simulink model "elp_elec_env"  (R2026b)
settings: Solver=VariableStepAuto
undefined symbols (not defined in the file or in its folder): P, Ts
libraries: simulink x1
settings Model: Creator=aomar  LastModifiedBy=aomar

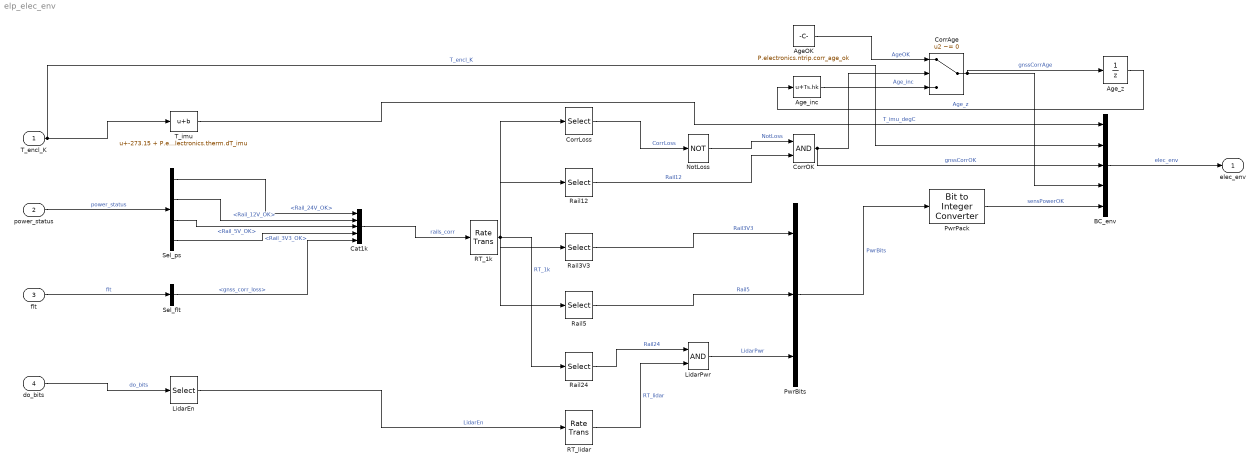
== system elp_elec_env ==
  T_encl_K : Inport  OutDataTypeStr=double  SampleTime=Ts.hk
  power_status : Inport  Port=2  OutDataTypeStr=Bus: Bus_PowerStatus  SampleTime=Ts.base
  flt : Inport  Port=3  OutDataTypeStr=Bus: Bus_FaultInject  SampleTime=Ts.base
  do_bits : Inport  Port=4  OutDataTypeStr=boolean  PortDimensions=32  SampleTime=Ts.ctrl
  AgeOK : Constant  Value=P.electronics.ntrip.corr_age_ok  OutDataTypeStr=double  SampleTime=Ts.hk
  Age_inc : Bias  Bias=Ts.hk  SaturateOnIntegerOverflow=off
  Age_z : UnitDelay  InitialCondition=P.electronics.ntrip.corr_age_ok  SampleTime=Ts.hk
  BC_env : BusCreator  Inputs=5  OutDataTypeStr=Bus: Bus_ElecEnv  NonVirtualBus=on
      settings: InheritFromInputs=off
  Cat1k : Concatenate  NumInputs=5
  CorrAge : Switch  Criteria=u2 ~= 0  SaturateOnIntegerOverflow=off  InputSameDT=off
  CorrLoss : Selector  InputPortWidth=5  IndexOptions=Index vector (dialog)  Indices=5  OutputSizes=1
  CorrOK : Logic  AllPortsSameDT=off  OutDataTypeStr=boolean
  LidarEn : Selector  InputPortWidth=32  IndexOptions=Index vector (dialog)  Indices=1 + P.electronics.do.lidar_pwr_en  OutputSizes=1
  LidarPwr : Logic  AllPortsSameDT=off  OutDataTypeStr=boolean
  NotLoss : Logic  Operator=NOT  Inputs=1  AllPortsSameDT=off  OutDataTypeStr=boolean
  PwrBits : Concatenate  NumInputs=3
  PwrPack : simulink/Logic and Bit Operations/Bit to Integer Converter  nbits=3  bitOrder=LSB first  signedOutputValues=Unsigned  outDtype=uint8  outDtypeSigned=Inherit via internal rule
      settings: LibrarySourceBlock=|
      | commutil2/Bit to Integer
      | Converter
  RT_1k : RateTransition  InitialCondition=false  OutPortSampleTime=Ts.hk
  RT_lidar : RateTransition  InitialCondition=false  OutPortSampleTime=Ts.hk
  Rail12 : Selector  InputPortWidth=5  IndexOptions=Index vector (dialog)  Indices=2  OutputSizes=1
  Rail24 : Selector  InputPortWidth=5  IndexOptions=Index vector (dialog)  Indices=1  OutputSizes=1
  Rail3V3 : Selector  InputPortWidth=5  IndexOptions=Index vector (dialog)  Indices=4  OutputSizes=1
  Rail5 : Selector  InputPortWidth=5  IndexOptions=Index vector (dialog)  Indices=3  OutputSizes=1
  Sel_flt : BusSelector  OutputSignals=gnss_corr_loss
  Sel_ps : BusSelector  OutputSignals=Rail_24V_OK,Rail_12V_OK,Rail_5V_OK,Rail_3V3_OK
  T_imu : Bias  Bias=-273.15 + P.electronics.therm.dT_imu  SaturateOnIntegerOverflow=off
  elec_env : Outport  OutDataTypeStr=Bus: Bus_ElecEnv
  wires:
  T_encl_K/1 -> T_imu/1, BC_env/2  "T_encl_K"
  power_status/1 -> Sel_ps/1  "power_status"
  flt/1 -> Sel_flt/1  "flt"
  do_bits/1 -> LidarEn/1  "do_bits"
  Sel_ps/1 -> Cat1k/1  "<Rail_24V_OK>"
  Sel_ps/2 -> Cat1k/2  "<Rail_12V_OK>"
  Sel_ps/3 -> Cat1k/3  "<Rail_5V_OK>"
  Sel_ps/4 -> Cat1k/4  "<Rail_3V3_OK>"
  Sel_flt/1 -> Cat1k/5  "<gnss_corr_loss>"
  T_imu/1 -> BC_env/1  "T_imu_degC"
  LidarEn/1 -> RT_lidar/1  "LidarEn"
  Cat1k/1 -> RT_1k/1  "rails_corr"
  RT_1k/1 -> Rail24/1, CorrLoss/1, Rail5/1, Rail12/1, Rail3V3/1  "RT_1k"
  CorrLoss/1 -> NotLoss/1  "CorrLoss"
  Rail12/1 -> CorrOK/2  "Rail12"
  Rail3V3/1 -> PwrBits/1  "Rail3V3"
  Rail5/1 -> PwrBits/2  "Rail5"
  Rail24/1 -> LidarPwr/1  "Rail24"
  RT_lidar/1 -> LidarPwr/2  "RT_lidar"
  NotLoss/1 -> CorrOK/1  "NotLoss"
  LidarPwr/1 -> PwrBits/3  "LidarPwr"
  PwrBits/1 -> PwrPack/1  "PwrBits"
  AgeOK/1 -> CorrAge/1  "AgeOK"
  CorrOK/1 -> CorrAge/2, BC_env/3  "gnssCorrOK"
  Age_inc/1 -> CorrAge/3  "Age_inc"
  CorrAge/1 -> BC_env/4, Age_z/1  "gnssCorrAge"
  PwrPack/1 -> BC_env/5  "sensPowerOK"
  BC_env/1 -> elec_env/1  "elec_env"
  Age_z/1 -> Age_inc/1  "Age_z"
